simulink model "AeroBenchSim_2019a"  (R2019a)
settings: Solver=VariableStepAuto  StartTime=0.0  StopTime=t_end  FixedStep=1/30.0  MaxStep=1/30  RelTol=1e-3  AbsTol=1e-6
InitFcn:
  | if ~exist("t_end", "var")
  |    fprintf("Please manually add the 'main' folder recursively to Matlab's PATH, set it as your current working directory, and run the SimConfig.m script before executing Simulink model.")
  | end
  | 
  | % Add simulink directories to MATLAB Path
  | %filepath=get_param(gcs, 'filename');
  | %path_sim = genpath(fileparts(filepath));
  | %addpath(path_sim);
  | 
  | % Configure workspace for sim
  | %SimConfig;
StopFcn:
  | %handleSimResults;
values from neighbouring files (symbols this model uses):
  ctrlLimits = F16.get_default_ctrl_srfc_limits()    [SimConfig.m]
  GCAS_config = GCAS.get_default_GCAS_config()    [SimConfig.m]
  K_lqr = getLqrControlGains(gain_str)    [SimConfig.m]
  v2_integrators = 0    [SimConfig.m]
  warnOn = false    [SimConfig.m]
  WF_config = WaypointFollower.get_default_WF_config()    [SimConfig.m]
undefined symbols (not defined in the file or in its folder): SIM_config, uequil, waypoints, x_f16_0, xequil
settings Model: Creator=HeidlaPT  LastModifiedBy=stan
settings DataIOCC: SaveFormat=StructureWithTime  SaveOutput=off  SignalLogging=off  DSMLogging=off  SaveTime=off  ReturnWorkspaceOutputs=off  TimeSaveName=t_out  OutputSaveName=x_f16_out  ReturnWorkspaceOutputsName=simout  LoggingIntervals=SIM_config.output_intervals
settings DebuggingCC: SFOutputUsedAsStateInMooreChartDiag=warning  ArithmeticOperatorsInVariantConditions=warning
settings SFSimCC: SimUseLocalCustomCode=off
settings RTWCC: RTWUseLocalCustomCode=off

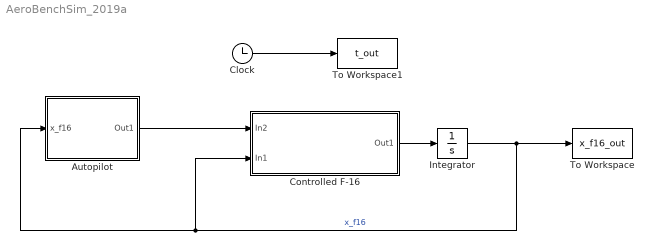
== system AeroBenchSim_2019a ==
  Autopilot : Subsystem
  Clock : Clock
  Controlled F-16 : Subsystem
  Integrator : Integrator  InitialCondition=x_f16_0
  To Workspace : ToWorkspace  VariableName=x_f16_out  SampleTime=SIM_config.t_sample
  To Workspace1 : ToWorkspace  VariableName=t_out  SampleTime=SIM_config.t_sample
  wires:
  Controlled F-16/1(Out1) -> Integrator/1
  Integrator/1 -> Autopilot/1(x_f16), Controlled F-16/2(In1), To Workspace/1  "x_f16"
  Autopilot/1(Out1) -> Controlled F-16/1(In2)
  Clock/1 -> To Workspace1/1

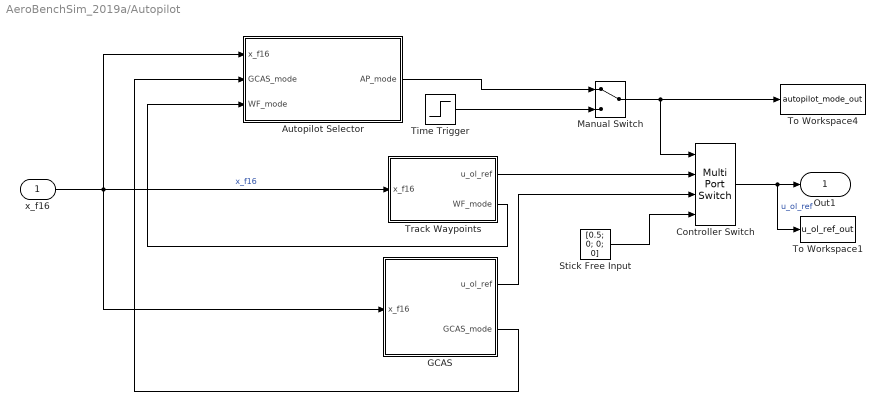
== system AeroBenchSim_2019a/Autopilot ==
  x_f16 : Inport
  Autopilot Selector : Stateflow chart  TreatAsAtomicUnit=on
  Controller Switch : MultiPortSwitch  DataPortOrder=Zero-based contiguous  Inputs=2  DataPortForDefault=Additional data port  DiagnosticForDefault=Warning  zeroidx=on  InputSameDT=on
  GCAS : Subsystem
  Manual Switch : ManualSwitch
  Stick Free Input : Constant  Value=[0.5; 0; 0; 0]  SampleTime=SIM_config.t_sample
  Time Trigger : Step  Time=15  SampleTime=0
  To Workspace1 : ToWorkspace  VariableName=u_ol_ref_out  SampleTime=SIM_config.t_sample
      settings: Save2DSignal=2-D array (concatenate along first dimension)
  To Workspace4 : ToWorkspace  VariableName=autopilot_mode_out  SampleTime=SIM_config.t_sample
      settings: Save2DSignal=2-D array (concatenate along first dimension)
  Track Waypoints : Subsystem
  Out1 : Outport
  wires:
  Time Trigger/1 -> Manual Switch/2
  x_f16/1 -> Autopilot Selector/1(x_f16), Track Waypoints/1(x_f16), GCAS/1(x_f16)  "x_f16"
  Stick Free Input/1 -> Controller Switch/4
  Controller Switch/1 -> To Workspace1/1, Out1/1  "u_ol_ref"
  Autopilot Selector/1(AP_mode) -> Manual Switch/1
  Manual Switch/1 -> Controller Switch/1, To Workspace4/1
  GCAS/1(u_ol_ref) -> Controller Switch/3
  Track Waypoints/1(u_ol_ref) -> Controller Switch/2
  GCAS/2(GCAS_mode) -> Autopilot Selector/2(GCAS_mode)
  Track Waypoints/2(WF_mode) -> Autopilot Selector/3(WF_mode)

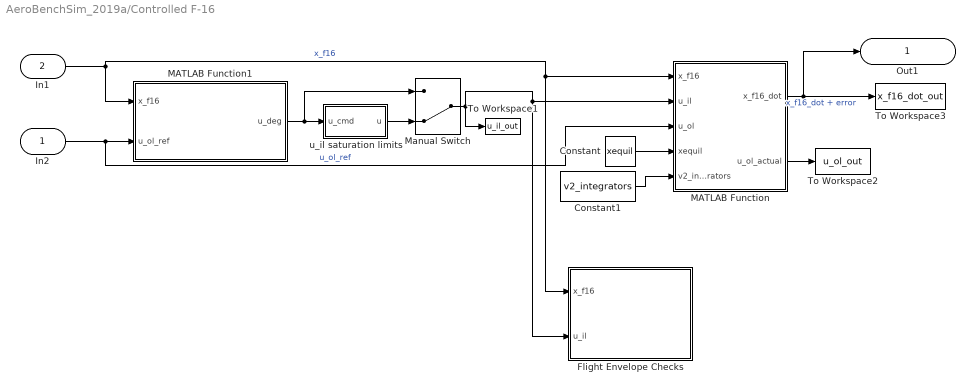
== system AeroBenchSim_2019a/Controlled F-16 ==
  In2 : Inport
  In1 : Inport  Port=2
  Constant : Constant  Value=xequil
  Constant1 : Constant  Value=v2_integrators
  Flight Envelope Checks : Stateflow chart  TreatAsAtomicUnit=on
  MATLAB Function : MATLAB Function  Tag=F-16  Description=Given aircraft state and raw control inputs, uses subf16_morelli to generate aircraft state derivatives  TreatAsAtomicUnit=on
  MATLAB Function1 : MATLAB Function  TreatAsAtomicUnit=on
  Manual Switch : ManualSwitch  CurrentSetting=0
  To Workspace1 : ToWorkspace  VariableName=u_il_out  SampleTime=SIM_config.t_sample
  To Workspace2 : ToWorkspace  VariableName=u_ol_out  SampleTime=SIM_config.t_sample
  To Workspace3 : ToWorkspace  VariableName=x_f16_dot_out  SampleTime=SIM_config.t_sample
  u_il saturation limits : Subsystem
  Out1 : Outport
  wires:
  In1/1 -> MATLAB Function1/1(x_f16), Flight Envelope Checks/1(x_f16), MATLAB Function/1(x_f16)  "x_f16"
  Manual Switch/1 -> To Workspace1/1, Flight Envelope Checks/2(u_il), MATLAB Function/2(u_il)
  MATLAB Function1/1(u_deg) -> u_il saturation limits/1(u_cmd), Manual Switch/1
  MATLAB Function/1(x_f16_dot) -> Out1/1, To Workspace3/1  "x_f16_dot + error"
  In2/1 -> MATLAB Function/3(u_ol), MATLAB Function1/2(u_ol_ref)  "u_ol_ref"
  MATLAB Function/2(u_ol_actual) -> To Workspace2/1
  u_il saturation limits/1(u) -> Manual Switch/2
  Constant/1 -> MATLAB Function/4(xequil)
  Constant1/1 -> MATLAB Function/5(v2_integrators)

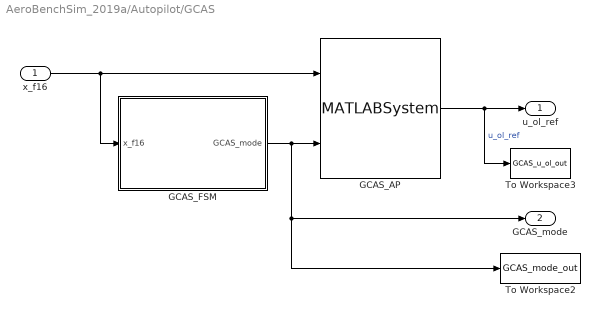
== system AeroBenchSim_2019a/Autopilot/GCAS ==
  x_f16 : Inport
  GCAS_AP : MATLABSystem  System=GCAS  SimulateUsing=Interpreted execution
      mask Type: GCAS
      mask Display:
      | disp('GCAS');
      | port_label('input',1,'x_f16');
      | port_label('input',2,'GCAS_mode');
      | port_label('output',1,'u_ol_ref');
  GCAS_FSM : Stateflow chart  TreatAsAtomicUnit=on
  To Workspace2 : ToWorkspace  VariableName=GCAS_mode_out  SampleTime=SIM_config.t_sample
      settings: Save2DSignal=2-D array (concatenate along first dimension)
  To Workspace3 : ToWorkspace  VariableName=GCAS_u_ol_out  SampleTime=SIM_config.t_sample
      settings: Save2DSignal=2-D array (concatenate along first dimension)
  u_ol_ref : Outport
  GCAS_mode : Outport  Port=2
  wires:
  GCAS_AP/1 -> To Workspace3/1, u_ol_ref/1  "u_ol_ref"
  x_f16/1 -> GCAS_AP/1, GCAS_FSM/1(x_f16)
  GCAS_FSM/1(GCAS_mode) -> To Workspace2/1, GCAS_mode/1, GCAS_AP/2

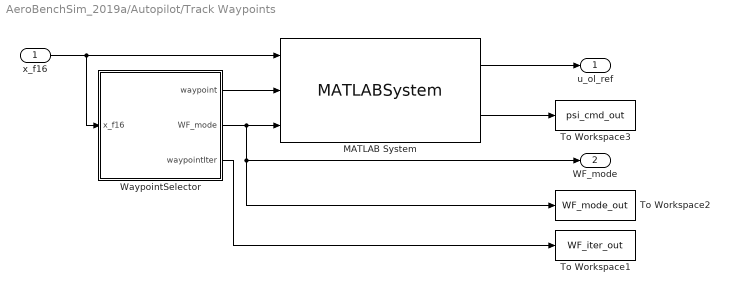
== system AeroBenchSim_2019a/Autopilot/Track Waypoints ==
  x_f16 : Inport
  MATLAB System : MATLABSystem  System=WaypointFollower  SimulateUsing=Interpreted execution
      mask Type: WaypointFollower
      mask Display:
      | disp('WaypointFollower');
      | port_label('input',1,'x_f16');
      | port_label('input',2,'waypoint');
      | port_label('input',3,'WF_mode');
      | port_label('output',1,'u_ol_ref');
      | port_label('output',2,'psi_cmd');
  To Workspace1 : ToWorkspace  VariableName=WF_iter_out  SampleTime=SIM_config.t_sample
      settings: Save2DSignal=2-D array (concatenate along first dimension)
  To Workspace2 : ToWorkspace  VariableName=WF_mode_out  SampleTime=SIM_config.t_sample
      settings: Save2DSignal=2-D array (concatenate along first dimension)
  To Workspace3 : ToWorkspace  VariableName=psi_cmd_out  SampleTime=SIM_config.t_sample
      settings: Save2DSignal=2-D array (concatenate along first dimension)
  WaypointSelector : Stateflow chart  TreatAsAtomicUnit=on
  u_ol_ref : Outport
  WF_mode : Outport  Port=2
  wires:
  x_f16/1 -> WaypointSelector/1(x_f16), MATLAB System/1
  MATLAB System/1 -> u_ol_ref/1
  WaypointSelector/2(WF_mode) -> To Workspace2/1, WF_mode/1, MATLAB System/3
  WaypointSelector/1(waypoint) -> MATLAB System/2
  WaypointSelector/3(waypointIter) -> To Workspace1/1
  MATLAB System/2 -> To Workspace3/1

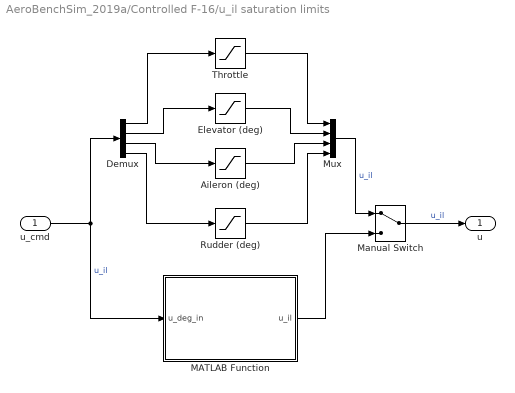
== system AeroBenchSim_2019a/Controlled F-16/u_il saturation limits ==
  u_cmd : Inport
  "Aileron (deg) " : Saturate  UpperLimit=ctrlLimits.aileronMax  LowerLimit=ctrlLimits.aileronMin
  Demux : Demux
  Elevator (deg) : Saturate  UpperLimit=ctrlLimits.elevatorMax  LowerLimit=ctrlLimits.elevatorMin
  MATLAB Function : MATLAB Function  TreatAsAtomicUnit=on
  Manual Switch : ManualSwitch
  Mux : Mux
  Rudder (deg) : Saturate  UpperLimit=ctrlLimits.rudderMax  LowerLimit=ctrlLimits.rudderMin
  Throttle : Saturate  UpperLimit=ctrlLimits.throttleMax  LowerLimit=ctrlLimits.throttleMin
  u : Outport  PortDimensions=4  LockScale=on
  wires:
  Demux/2 -> Elevator (deg)/1
  Demux/4 -> Rudder (deg)/1
  Mux/1 -> Manual Switch/1  "u_il"
  Demux/1 -> Throttle/1
  Elevator (deg)/1 -> Mux/2
  u_cmd/1 -> Demux/1, MATLAB Function/1(u_deg_in)  "u_il"
  "Aileron (deg) "/1 -> Mux/3
  Rudder (deg)/1 -> Mux/4
  Throttle/1 -> Mux/1
  Demux/3 -> "Aileron (deg) "/1
  Manual Switch/1 -> u/1  "u_il"
  MATLAB Function/1(u_il) -> Manual Switch/2

== matlab function AeroBenchSim_2019a/Controlled F-16/MATLAB Function1 ==
  data: x_f16 input; u_deg output; u_ol_ref input; xequil parameter; uequil parameter; K_lqr parameter
function u_deg  = LQR_controller(...
    x_f16, u_ol_ref, xequil, uequil, K_lqr)
%LQR_CONTROLLER Given x_f16, ref control, and workspace vars, evaluates
%u_deg (4x1)

%Declare function as extrinsic
coder.extrinsic('getInnerLoopControl');

u_deg = zeros(4,1);
u_deg = getInnerLoopControl(x_f16, u_ol_ref, xequil, uequil, K_lqr);

end

== matlab function AeroBenchSim_2019a/Controlled F-16/MATLAB Function ==
  data: x_f16 input; u_il input size=[4 1]; x_f16_dot output; u_ol_actual output; u_ol input; xequil input; v2_integrators input
function [x_f16_dot, u_ol_actual] = F16_plant(x_f16, u_il, u_ol, xequil, v2_integrators)

%Declare function as extrinsic
coder.extrinsic('subf16_morelli');

% Preallocate so simulink knows size of outputs
% Note: alternate method is to specify using "Edit Data" in menu
x_f16_dot = zeros(size(x_f16));
u_ol_actual = zeros(4,1);

x_f16_delta = x_f16 - [xequil; 0; 0; 0];

[x_f16_dot, u_ol_actual] = subf16_morelli(x_f16, u_il, x_f16_delta, v2_integrators);

%fprintf("integrator calc:\n");
%u_ol_actual(1:3)
%u_ol(1:3)

% Append error states for integration
x_f16_dot(14:16) = u_ol_actual(1:3) - u_ol(1:3); 

%fprintf("\nState:\n");
%for i=1:16
%   fprintf("%.9f\n", x_f16(i));
%end

%fprintf("u_ol:\n");
%for i=1:3
%   fprintf("%.9f\n", u_ol(i));
%end

%fprintf("---\nDer:\n");
%for i=1:16
%   fprintf("%.9f\n", x_f16_dot(i));
%end

== stateflow chart AeroBenchSim_2019a/Controlled F-16/Flight Envelope Checks ==
  settings: executeAtInitialization=1
  state CRASH
    entry: fprintf('CRASHED\n'),
    % F16_crashed = true;
  state SAFE
    entry: fprintf('In flight envelope\n');
  state OUT_OF_MODEL_RANGE
    entry: fprintf('Model no longer valid, stopping sim\n')
    stopSimulink();
  state STALL
    entry: fprintf('STALLED\n'),
    % F16_stalled = true;
  state OVERSTRESS [commented out]
    entry: fprintf('OVERSTRESSED\n'),
    % F16_overstressed = true;
  (default) -> SAFE
  SAFE -> CRASH [order 1] : [~F16.is_in_altitude_limits(flightLimits, x_f16)]
  STALL -> OUT_OF_MODEL_RANGE
  CRASH -> OUT_OF_MODEL_RANGE
  SAFE -> OVERSTRESS [commented out] : [~F16.is_in_Nz_limits(flightLimits, x_f16)]
  SAFE -> STALL [order 2] : [~F16.is_in_alpha_limits(flightLimits, x_f16)]
  data: x_f16 input; u_il input; flightLimits parameter

== matlab function AeroBenchSim_2019a/Controlled F-16/u_il saturation limits/MATLAB Function ==
  data: u_deg_in input; u_il output; ctrlLimits parameter; warnOn parameter
function u_il = control_saturation(u_deg_in, ctrlLimits, warnOn)

u_il = applyCtrlSatLimits(u_deg_in,ctrlLimits,warnOn);

end

== stateflow chart AeroBenchSim_2019a/Autopilot/GCAS/GCAS_FSM ==
  settings: executeAtInitialization=1
  state ROLL_LEVEL
    entry: GCAS_mode = 1;
    printGCASUpdate();
  state SAFE
    entry: GCAS_mode = 0;
    printGCASUpdate();
  state PULL_UP
    entry: GCAS_mode = 2;
    printGCASUpdate();
  (default) -> (junction 45)
  (junction 45) -> SAFE [order 2]
  (junction 45) -> ROLL_LEVEL [order 1] : [GCAS_starts_on]
  SAFE -> ROLL_LEVEL : [~GCAS.isNoseHighEnough(x_f16, GCAS_config) && ...
      | ~GCAS.isAboveFlightDeck(x_f16, GCAS_config)]
  PULL_UP -> SAFE : [GCAS.isNoseHighEnough(x_f16, GCAS_config) && ...
      | after(GCAS_config.min_pull_time, sec)]
  ROLL_LEVEL -> PULL_UP : [GCAS.isRollRateLow(x_f16, GCAS_config) && ...
      | GCAS.areWingsLevel(x_f16, GCAS_config)]
  data: x_f16 input; GCAS_config parameter; GCAS_mode output; GCAS_starts_on constant double =GCAS_starts_on
  data GCAS_config settings: description=|
      | defines GCAS constants:
      | eps_p
      | eps_phi
      | path_goal
  function printGCASUpdate:
    | function printGCASUpdate
    | % Prints update to Simulink console
    | 
    | fprintf('Entering GCAS_mode %f at time %.6f\n', round(GCAS_mode), t);
    |     
    | end

== stateflow chart AeroBenchSim_2019a/Autopilot/Track Waypoints/WaypointSelector ==
  settings: executeAtInitialization=1
  state TRACK_TO_WAYPOINT
    entry: waypoint = waypoints(waypointIter,:);
    WF_mode = 0;
    exit: printWaypointUpdate();
    waypointIter = waypointIter + 1;
  state COMPLETE
    entry: WF_mode = 1;
    waypoint = waypoints(waypointIter - 1,:);
    fprintf('Waypoint navigation complete\n');
  (default) -> TRACK_TO_WAYPOINT
  TRACK_TO_WAYPOINT -> (junction 28) : [waypointIter > size(waypoints,1) || ...
      | closeEnoughToWaypoint()]
  (junction 28) -> COMPLETE [order 2]
  (junction 28) -> TRACK_TO_WAYPOINT [order 1] : [waypointIter < size(waypoints,1)]
  data: isCloseEnough function_output; waypoint output; WF_mode output; x_f16 input; waypoints parameter; WF_config parameter; waypointIter output int8 [1..] =int8(1)
  function isCloseEnough = closeEnoughToWaypoint:
    | function isCloseEnough = closeEnoughToWaypoint()
    | 
    | [~,~,~,~,slant_range] = WaypointFollower.getWaypointData(x_f16,waypoint);  
    |             
    | isCloseEnough = slant_range < WF_config.WP_RANGE_THRESHOLD;
    |     
    | % isCloseEnough = horiz_range < WF_config.WP_VERT_RANGE_THRESHOLD && ...
    | %     vert_range < WF_config.WP_HORIZ_RANGE_THRESHOLD;
    | 
    | end
  function printWaypointUpdate:
    | function printWaypointUpdate()
    | % Prints update to Simulink console
    | 
    | fprintf('Waypoint Iter: %d at time %.5f, Target: [ %6.0f E, %6.0f N, %6.0f U ]\n', ...
    |     waypointIter, t, waypoint(1), waypoint(2), waypoint(3));
    |     
    | end

== stateflow chart AeroBenchSim_2019a/Autopilot/Autopilot Selector ==
  settings: executeAtInitialization=1
  state USE_GCAS_AP
    entry: AP_mode  = 1;
    fprintf('Activate GCAS\n');
  state USE_WF_AP
    entry: AP_mode = 0;
    fprintf('Follow Waypoints\n');
  state WF_COMPLETE
    entry:  fprintf('Waypoint Following Complete\n');
  state SIM_COMPLETE
    entry: stopSimulink();
  (default) -> (junction 48)
  (junction 48) -> USE_WF_AP [order 2]
  (junction 48) -> USE_GCAS_AP [order 1] : [GCAS_starts_on]
  USE_GCAS_AP -> USE_WF_AP : [GCAS_mode == 0]
  USE_WF_AP -> USE_GCAS_AP [order 2] : [(x_f16(12) < GCAS_config.FLIGHT_DECK) ...
      | &&  ~GCAS.isNoseHighEnough(x_f16, GCAS_config)]
  WF_COMPLETE -> USE_GCAS_AP [order 2] : [GCAS_mode ~= 0]
  USE_WF_AP -> WF_COMPLETE [order 1] : [WF_mode == 1]
  WF_COMPLETE -> SIM_COMPLETE [order 1] : [SIM_config.auto_stop && ...
      | after(SIM_config.auto_stop_delay, sec)]
  data: x_f16 input; AP_mode output; GCAS_config parameter; GCAS_mode input; WF_mode input; SIM_config parameter; GCAS_starts_on constant double =GCAS_starts_on
